simulink model "PMSMHighFrequencyPlantTest"  (R2026b)
settings: Solver=ode4  StopTime=hfPlantTestCfg.Duration  FixedStep=hfPlantTestCfg.PlantStep
PostLoadFcn:
  | addpath(fullfile(fileparts(get_param(bdroot,'FileName')),'..','build_process'));initialize_hf_plant_test(bdroot);
model workspace (MAT data in the model file):
  hfPlantCfg.Rs = 0.5
  hfPlantCfg.Ld = 0.001
  hfPlantCfg.Lq = 0.0015
  hfPlantCfg.Flux = 0.035
  hfPlantCfg.PolePairs = 4
  hfPlantCfg.J = 0.0005
  hfPlantCfg.B = 0.0001
  hfPlantCfg.Id0 = 0
  hfPlantCfg.Iq0 = 0
  hfPlantCfg.Speed0 = 0
  hfPlantCfg.Position0 = 0
  hfPlantCfg.SaturationDepth = 0.25
  hfPlantCfg.SaturationCurrent = 1
  hfPlantCfg.CrossInductance = 0
  hfPlantCfg.MechanicalEnabled = 1
  hfPlantCfg.Settings = [0.5; 0.001; 0.0015; 0.035; 4; 0.0005; 0.0001; 0.25; 1; 0; 1]
  hfPlantCfg.InitialState = [0; 0; 0; 0]
  hfPlantTestCfg.Ts = 5e-05
  hfPlantTestCfg.PlantStep = 2.5e-06
  hfPlantTestCfg.Duration = 0.1
  hfPlantTestCfg.PulseVoltage = 4
  hfPlantTestCfg.PositiveStart = 0.02
  hfPlantTestCfg.NegativeStart = 0.065
  hfPlantTestCfg.PulseWidth = 0.001
  hfPlantTestCfg.VoltageAxis = 0
  hfPlantTestCfg.LoadTorque = 0
  testStim.time = [0 5e-05 0.0001 0.00015 0.0002 0.00025 0.0003 0.00035 0.0004 0.00045 0.0005 0.00055 ... (2001 elements, 2001x1)]
  testStim.signals.values = [0 0 0 0 0 0 0 0 0 0 0 0 ... (6003 elements, 2001x3)]
  testStim.signals.dimensions = 3
libraries: PMSMHighFrequencyPlant x1
settings Model: Creator=24322  LastModifiedBy=24322

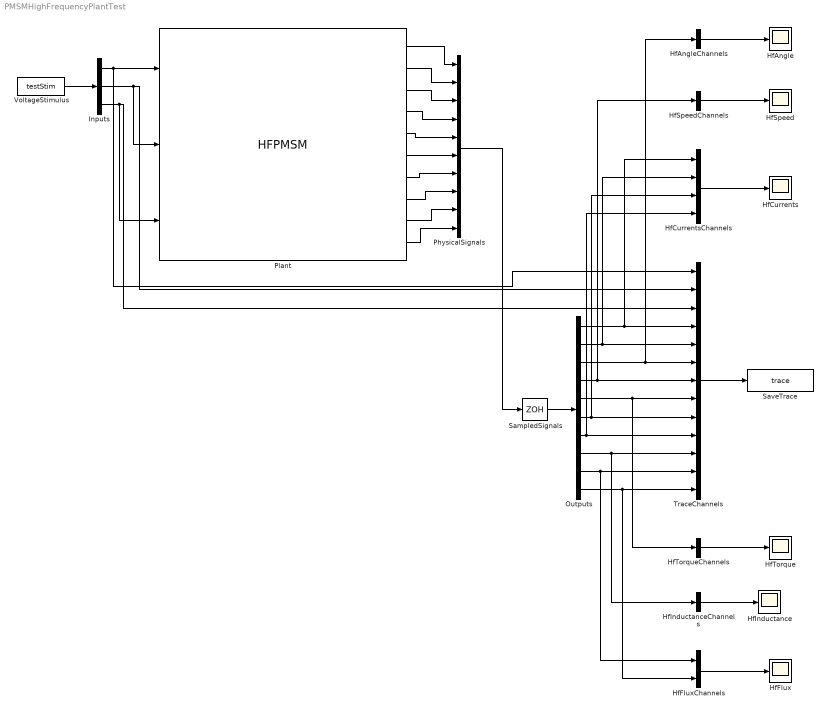
== system PMSMHighFrequencyPlantTest ==
  HfAngle : Scope
  HfAngleChannels : Mux  Inputs=1
  HfCurrents : Scope
  HfCurrentsChannels : Mux
  HfFlux : Scope
  HfFluxChannels : Mux  Inputs=2
  HfInductance : Scope
  HfInductanceChannels : Mux  Inputs=1
  HfSpeed : Scope
  HfSpeedChannels : Mux  Inputs=1
  HfTorque : Scope
  HfTorqueChannels : Mux  Inputs=1
  Inputs : Demux  Outputs=3
  Outputs : Demux  Outputs=10
  PhysicalSignals : Mux  Inputs=10
  Plant : PMSMHighFrequencyPlant/HFPMSM  cfg=hfPlantCfg
  SampledSignals : ZeroOrderHold  SampleTime=hfPlantTestCfg.Ts
  SaveTrace : ToWorkspace  VariableName=trace  SaveFormat=Structure With Time  SampleTime=-1
  TraceChannels : Mux  Inputs=13
  VoltageStimulus : FromWorkspace  VariableName=testStim  SampleTime=hfPlantTestCfg.Ts  Interpolate=off  OutputAfterFinalValue=Holding final value
  wires:
  HfInductanceChannels/1 -> HfInductance/1
  HfFluxChannels/1 -> HfFlux/1
  HfTorqueChannels/1 -> HfTorque/1
  HfSpeedChannels/1 -> HfSpeed/1
  HfAngleChannels/1 -> HfAngle/1
  HfCurrentsChannels/1 -> HfCurrents/1
  Outputs/10 -> TraceChannels/13, HfFluxChannels/2
  Plant/10 -> PhysicalSignals/10
  Outputs/9 -> TraceChannels/12, HfFluxChannels/1
  Plant/9 -> PhysicalSignals/9
  Outputs/8 -> TraceChannels/11, HfInductanceChannels/1
  Plant/8 -> PhysicalSignals/8
  Outputs/7 -> TraceChannels/10, HfCurrentsChannels/4
  Plant/7 -> PhysicalSignals/7
  Outputs/6 -> TraceChannels/9, HfCurrentsChannels/3
  Plant/6 -> PhysicalSignals/6
  Outputs/5 -> TraceChannels/8, HfTorqueChannels/1
  Plant/5 -> PhysicalSignals/5
  Outputs/4 -> TraceChannels/7, HfSpeedChannels/1
  Plant/4 -> PhysicalSignals/4
  Outputs/3 -> TraceChannels/6, HfAngleChannels/1
  Plant/3 -> PhysicalSignals/3
  Outputs/2 -> TraceChannels/5, HfCurrentsChannels/2
  Plant/2 -> PhysicalSignals/2
  Outputs/1 -> TraceChannels/4, HfCurrentsChannels/1
  Plant/1 -> PhysicalSignals/1
  Inputs/3 -> Plant/3, TraceChannels/3
  Inputs/2 -> Plant/2, TraceChannels/2
  Inputs/1 -> Plant/1, TraceChannels/1
  TraceChannels/1 -> SaveTrace/1
  SampledSignals/1 -> Outputs/1
  PhysicalSignals/1 -> SampledSignals/1
  VoltageStimulus/1 -> Inputs/1
